simulink model "FMT_MotorRHS"  (R2026b)
settings: Solver=FixedStepDiscrete  StopTime=2  FixedStep=0.0005
undefined symbols (not defined in the file): MotorKf, MotorMaxN, MotorTau
settings Model: DataDictionary=Flight_Parameters.sldd  Creator=26718  LastModifiedBy=26718

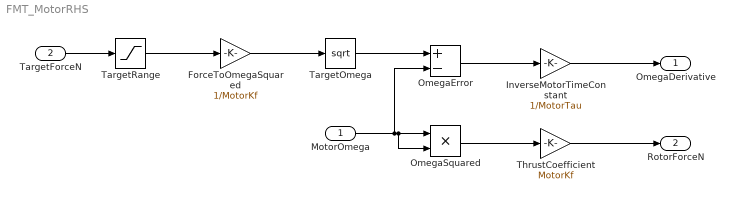
== system FMT_MotorRHS ==
  MotorOmega : Inport  OutDataTypeStr=double  PortDimensions=4
  TargetForceN : Inport  Port=2  OutDataTypeStr=double  PortDimensions=4
  ForceToOmegaSquared : Gain  Gain=1/MotorKf
  InverseMotorTimeConstant : Gain  Gain=1/MotorTau
  OmegaError : Sum  Inputs=+-
  OmegaSquared : Product  Inputs=**
  TargetOmega : Sqrt
  TargetRange : Saturate  UpperLimit=MotorMaxN  LowerLimit=0
  ThrustCoefficient : Gain  Gain=MotorKf
  OmegaDerivative : Outport
  RotorForceN : Outport  Port=2
  wires:
  ThrustCoefficient/1 -> RotorForceN/1
  OmegaSquared/1 -> ThrustCoefficient/1
  InverseMotorTimeConstant/1 -> OmegaDerivative/1
  OmegaError/1 -> InverseMotorTimeConstant/1
  MotorOmega/1 -> OmegaSquared/1, OmegaSquared/2, OmegaError/2
  TargetOmega/1 -> OmegaError/1
  ForceToOmegaSquared/1 -> TargetOmega/1
  TargetRange/1 -> ForceToOmegaSquared/1
  TargetForceN/1 -> TargetRange/1
